simulink model "Hinf_nonlinear_sim"  (R2026a)
settings: Solver=VariableStepAuto
InitFcn:
  | seaDir=fileparts(get_param(bdroot,'FileName'));if isfile(fullfile(seaDir,'..','collaudo_simulink.m')),addpath(fullfile(seaDir,'..'));else,addpath(fullfile(seaDir,'..','..','File_di_Funzioni_Progetto-Accorpati'));end;collaudo_simulink(bdroot);
undefined symbols (not defined in the file): Ak1, Ak2, Bk1, Bk2, Ck1, Ck2, Dk1, Dk2, taubar, xbar
libraries: cstblocks_lti x7
settings Model: Creator=rebec  LastModifiedBy=rebec

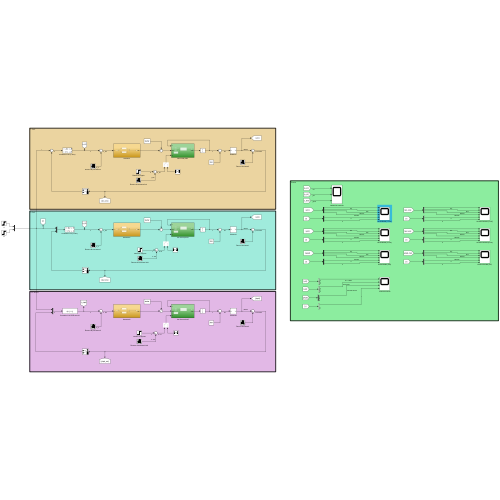
[thumbnail: Simulink's stored preview of the top-level diagram]
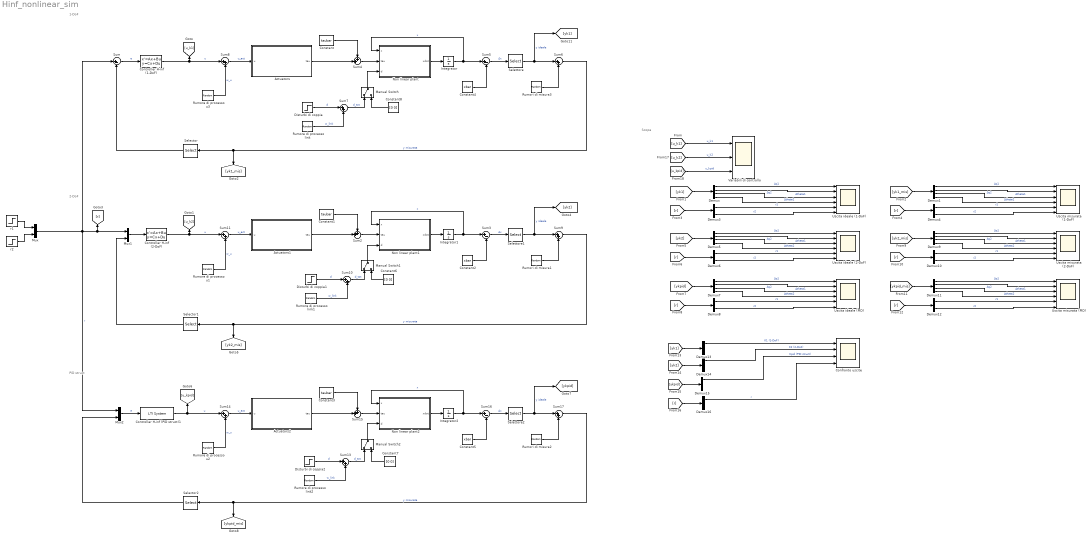
== system Hinf_nonlinear_sim ==
  note: Scope
  note: 2-DoF
  note: PID struct
  note: 1-DoF
  Actuators : Subsystem
  Actuators1 : Subsystem
  Actuators2 : Subsystem
  Confronto uscite : Scope  NumInputPorts=4
      settings: Title=Uscite  ActiveDisplayYMinimum=-0.27933944069600969  ActiveDisplayYMaximum=0.21495071578525782  YLabel=y (rad)  DataLoggingVariableName=ScopeData7
  Constant : Constant  Value=taubar
  Constant1 : Constant  Value=taubar
  Constant2 : Constant  Value=xbar
  Constant3 : Constant  Value=taubar
  Constant4 : Constant  Value=xbar
  Constant5 : Constant  Value=xbar
  Constant6 : Constant  Value=[0 0]
  Constant7 : Constant  Value=[0 0]
  Constant8 : Constant  Value=[0 0]
  Controller H-inf (1-DoF) : StateSpace  A=Ak1  B=Bk1  C=Ck1  D=Dk1  InitialCondition=0
  Controller H-inf (2-DoF) : StateSpace  A=Ak2  B=Bk2  C=Ck2  D=Dk2  InitialCondition=0
  Controller H-inf (PID struct)1 : cstblocks_lti/LTI System  sys=Kpid  IC=[]  PadeOrder=0
      settings: LibrarySourceBlock=cstblocks/LTI System
  Demux{,1,5,7,9,11,13..15} (9 alike) : Demux
  Demux{3..4,6,8,10,12,16} (7 alike) : Demux  Outputs=2
  Disturbi di coppia : Step  Time=[1 1]  InitialValue=[0 0]  FinalValue=[0.5 0]  SampleTime=0
  Disturbi di coppia1 : Step  Time=[1 1]  InitialValue=[0 0]  FinalValue=[0.5 0]  SampleTime=0
  Disturbi di coppia2 : Step  Time=[1 1]  InitialValue=[0 0]  FinalValue=[0.5 0]  SampleTime=0
  Integrator : Integrator  InitialCondition=xbar
  Integrator1 : Integrator  InitialCondition=xbar
  Integrator2 : Integrator  InitialCondition=xbar
  Manual Switch : ManualSwitch
  Manual Switch1 : ManualSwitch
  Manual Switch2 : ManualSwitch
  Mux : Mux  Inputs=2
  Mux1 : Mux  Inputs=2
  Mux2 : Mux  Inputs=2
  Non linear plant : Subsystem
  Non linear plant1 : Subsystem
  Non linear plant2 : Subsystem
  Rumore di processo link : RandomNumber  Mean=[0 0]  Variance=[0.01 0.01]  Seed=20260826  SampleTime=0.002
  Rumore di processo link1 : RandomNumber  Mean=[0 0]  Variance=[0.01 0.01]  Seed=20260826  SampleTime=0.002
  Rumore di processo link2 : RandomNumber  Mean=[0 0]  Variance=[0.01 0.01]  Seed=20260826  SampleTime=0.002
  Rumore di processo u1 : RandomNumber  Mean=[0 0]  Variance=[0.01 0.01]  Seed=20260826  SampleTime=0.002
  Rumore di processo u2 : RandomNumber  Mean=[0 0]  Variance=[0.01 0.01]  Seed=20260826  SampleTime=0.002
  Rumore di processo u3 : RandomNumber  Mean=[0 0]  Variance=[0.01 0.01]  Seed=20260826  SampleTime=0.002
  Rumori di misura1 : RandomNumber  Mean=[0 0 0 0]  Variance=[(0.05*pi/180)^2 (0.05*pi/180)^2 (0.05*pi/180)^2 (0.05*pi/180)^2]  Seed=20260826  SampleTime=0.002
  Rumori di misura2 : RandomNumber  Mean=[0 0 0 0]  Variance=[(0.05*pi/180)^2 (0.05*pi/180)^2 (0.05*pi/180)^2 (0.05*pi/180)^2]  Seed=20260826  SampleTime=0.002
  Rumori di misura3 : RandomNumber  Mean=[0 0 0 0]  Variance=[(0.05*pi/180)^2 (0.05*pi/180)^2 (0.05*pi/180)^2 (0.05*pi/180)^2]  Seed=20260826  SampleTime=0.002
  Selector : Selector  InputPortWidth=4  IndexOptions=Index vector (dialog)  Indices=[1 2]  OutputSizes=1
  Selector1 : Selector  InputPortWidth=4  IndexOptions=Index vector (dialog)  Indices=[1 2]  OutputSizes=1
  Selector2 : Selector  InputPortWidth=4  IndexOptions=Index vector (dialog)  Indices=[1 2]  OutputSizes=1
  Selettore : Selector  InputPortWidth=8  IndexOptions=Index vector (dialog)  Indices=[1 2 5 6]  OutputSizes=1
  Selettore1 : Selector  InputPortWidth=8  IndexOptions=Index vector (dialog)  Indices=[1 2 5 6]  OutputSizes=1
  Selettore2 : Selector  InputPortWidth=8  IndexOptions=Index vector (dialog)  Indices=[1 2 5 6]  OutputSizes=1
  Sum{,3,5,16} (4 alike) : Sum  Inputs=|+-
  Sum{6..11,13..14,17} (9 alike) : Sum  Inputs=|++
  Sum15 : Sum  Inputs=++|
  Sum2 : Sum  Inputs=++|
  Sum4 : Sum  Inputs=++|
  Uscita ideale (1-DoF) : Scope  NumInputPorts=6
      settings: Title=Uscita ideale (1-DoF)  ActiveDisplayYMinimum=-0.57230265617122578  ActiveDisplayYMaximum=0.50667076569906444  YLabel=y (rad)
  Uscita ideale (2-DoF) : Scope  NumInputPorts=6
      settings: Title=Uscita ideale (2-DoF)  ActiveDisplayYMinimum=-0.30624818665705794  ActiveDisplayYMaximum=0.42404349584753864  YLabel=y (rad)  DataLoggingVariableName=ScopeData3
  Uscita ideale (PID) : Scope  NumInputPorts=6
      settings: Title=Uscita ideale (PID struct)  ActiveDisplayYMinimum=-0.20967372209927659  ActiveDisplayYMaximum=0.28461643438199091  YLabel=y (rad)  DataLoggingVariableName=ScopeData4
  Uscita misurata (1-DoF) : Scope  NumInputPorts=6
      settings: Title=Uscita misurata (1-DoF)  ActiveDisplayYMinimum=-0.57230265617122578  ActiveDisplayYMaximum=0.50667076569906444  YLabel=y_m_i_s (rad)
  Uscita misurata (2-DoF) : Scope  NumInputPorts=6
      settings: Title=Uscita misurata (2-DoF)  ActiveDisplayYMinimum=-0.33288828600734088  ActiveDisplayYMaximum=0.43391798062248577  YLabel=y_m_i_s (rad)  DataLoggingVariableName=ScopeData5
  Uscita misurata (PID) : Scope  NumInputPorts=6
      settings: Title=Uscita misurata (PID struct)  ActiveDisplayYMinimum=-0.20967372209927659  ActiveDisplayYMaximum=0.28461643438199091  YLabel=y_m_i_s (rad)  DataLoggingVariableName=ScopeData6
  Variabili di controllo : Scope  NumInputPorts=3
      settings: ActiveDisplayString=3  Title=PID struct  ActiveDisplayYMinimum=-392.20426405655667  ActiveDisplayYMaximum=429.18075042306987  YLabel=u_k_p_i_d (Nm)  DataLoggingVariableName=ScopeData10
  r1 : Step  FinalValue=5*pi/180  SampleTime=0
  r2 : Step  FinalValue=0  SampleTime=0
  wires:
  Demux10/1 -> Uscita misurata (2-DoF)/5  "r1"
  Demux8/1 -> Uscita ideale (PID)/5  "r1"
  Demux8/2 -> Uscita ideale (PID)/6  "r2"
  Demux9/4 -> Uscita misurata (2-DoF)/4  "Δtheta2"
  Demux4/1 -> Uscita misurata (1-DoF)/5  "r1"
  [u_kpid] -> Variabili di controllo/3  "u_kpid"
  Demux15/1 -> Confronto uscite/3  "Kpid (PID struct)"
  r1/1 -> Mux/1
  Demux3/2 -> Uscita ideale (1-DoF)/6  "r2"
  Selector/1 -> Sum/2
  Demux7/3 -> Uscita ideale (PID)/3  "Δtheta1"
  Demux5/3 -> Uscita ideale (2-DoF)/3  "Δtheta1"
  Demux5/2 -> Uscita ideale (2-DoF)/2  "Δq2"
  Demux11/3 -> Uscita misurata (PID)/3  "Δtheta1"
  Demux7/4 -> Uscita ideale (PID)/4  "Δtheta2"
  Demux1/2 -> Uscita misurata (1-DoF)/2  "Δq2"
  Demux1/1 -> Uscita misurata (1-DoF)/1  "Δq1"
  [r] -> Demux10/1
  [yk1_mis] -> Demux1/1
  [r] -> Demux16/1
  [ykpid] -> Demux15/1
  Demux9/2 -> Uscita misurata (2-DoF)/2  "Δq2"
  Controller H-inf (1-DoF)/1 -> Sum8/1, [u_k1]  "u"
  Demux11/4 -> Uscita misurata (PID)/4  "Δtheta2"
  [u_k1] -> Variabili di controllo/1  "u_k1"
  Demux/3 -> Uscita ideale (1-DoF)/3  "Δtheta1"
  Demux11/1 -> Uscita misurata (PID)/1  "Δq1"
  [r] -> Demux3/1
  Demux7/2 -> Uscita ideale (PID)/2  "Δq2"
  Demux/2 -> Uscita ideale (1-DoF)/2  "Δq2"
  Demux9/3 -> Uscita misurata (2-DoF)/3  "Δtheta1"
  [yk2] -> Demux5/1
  [yk2_mis] -> Demux9/1
  Demux14/1 -> Confronto uscite/2  "K2 (2-DoF)"
  [yk1] -> Demux/1
  [ykpid] -> Demux7/1
  Demux5/4 -> Uscita ideale (2-DoF)/4  "Δtheta2"
  Demux/1 -> Uscita ideale (1-DoF)/1  "Δq1"
  r2/1 -> Mux/2
  Demux6/1 -> Uscita ideale (2-DoF)/5  "r1"
  Demux3/1 -> Uscita ideale (1-DoF)/5  "r1"
  Demux4/2 -> Uscita misurata (1-DoF)/6  "r2"
  [r] -> Demux12/1
  [r] -> Demux6/1
  [r] -> Demux8/1
  Demux9/1 -> Uscita misurata (2-DoF)/1  "Δq1"
  Mux/1 -> Mux2/1, Mux1/1, [r], Sum/1  "r"
  Demux1/3 -> Uscita misurata (1-DoF)/3  "Δtheta1"
  Sum/1 -> Controller H-inf (1-DoF)/1  "e"
  Demux13/1 -> Confronto uscite/1  "K1 (1-DoF)"
  Demux6/2 -> Uscita ideale (2-DoF)/6  "r2"
  [yk2] -> Demux14/1
  Demux16/1 -> Confronto uscite/4  "r"
  Demux/4 -> Uscita ideale (1-DoF)/4  "Δtheta2"
  [r] -> Demux4/1
  [yk1] -> Demux13/1
  Demux12/1 -> Uscita misurata (PID)/5  "r1"
  [ykpid_mis] -> Demux11/1
  Demux7/1 -> Uscita ideale (PID)/1  "Δq1"
  Demux5/1 -> Uscita ideale (2-DoF)/1  "Δq1"
  Demux10/2 -> Uscita misurata (2-DoF)/6  "r2"
  Demux1/4 -> Uscita misurata (1-DoF)/4  "Δtheta2"
  Demux11/2 -> Uscita misurata (PID)/2  "Δq2"
  Demux12/2 -> Uscita misurata (PID)/6  "r2"
  [u_k2] -> Variabili di controllo/2  "u_k2"
  Actuators/1(tau) -> Sum4/2
  Disturbi di coppia/1 -> Sum7/1  "d"
  Sum4/1 -> Non linear plant/2(tau)
  Constant/1 -> Sum4/1
  Selettore/1 -> Sum6/1, [yk1]  "y ideale"
  Constant4/1 -> Sum5/2
  Integrator/1 -> Non linear plant/1(x), Sum5/1  "x"
  Sum5/1 -> Selettore/1  "Δx"
  Sum8/1 -> Actuators/1(u)  "u_act"
  Non linear plant/1(xdot) -> Integrator/1
  Sum6/1 -> [yk1_mis], Selector/1  "y misurata"
  Rumore di processo link/1 -> Sum7/2  "w_link"
  Sum9/1 -> [yk2_mis], Selector1/1  "y misurata"
  Controller H-inf (2-DoF)/1 -> Sum11/1, [u_k2]  "u"
  Selector1/1 -> Mux1/2
  Rumore di processo link1/1 -> Sum10/2  "w_link"
  Sum11/1 -> Actuators1/1(u)  "u_act"
  Non linear plant1/1(xdot) -> Integrator1/1
  Sum3/1 -> Selettore1/1  "Δx"
  Selettore1/1 -> Sum9/1, [yk2]  "y ideale"
  Constant2/1 -> Sum3/2
  Sum2/1 -> Non linear plant1/2(tau)
  Integrator1/1 -> Non linear plant1/1(x), Sum3/1  "x"
  Actuators1/1(tau) -> Sum2/2
  Constant1/1 -> Sum2/1
  Disturbi di coppia1/1 -> Sum10/1  "d"
  Constant3/1 -> Sum15/1
  Actuators2/1(tau) -> Sum15/2
  Disturbi di coppia2/1 -> Sum13/1  "d"
  Selettore2/1 -> Sum17/1, [ykpid]  "y ideale"
  Sum15/1 -> Non linear plant2/2(tau)
  Constant5/1 -> Sum16/2
  Mux2/1 -> Controller H-inf (PID struct)1/1  "e"
  Sum16/1 -> Selettore2/1  "Δx"
  Controller H-inf (PID struct)1/1 -> Sum14/1, [u_kpid]  "u"
  Selector2/1 -> Mux2/2
  Rumore di processo link2/1 -> Sum13/2  "w_link"
  Sum14/1 -> Actuators2/1(u)  "u_act"
  Sum17/1 -> [ykpid_mis], Selector2/1  "y misurata"
  Non linear plant2/1(xdot) -> Integrator2/1
  Integrator2/1 -> Non linear plant2/1(x), Sum16/1  "x"
  Mux1/1 -> Controller H-inf (2-DoF)/1
  Manual Switch/1 -> Non linear plant/3(d)
  Sum7/1 -> Manual Switch/1  "d_tot"
  Constant8/1 -> Manual Switch/2
  Manual Switch1/1 -> Non linear plant1/3(d)
  Sum10/1 -> Manual Switch1/1  "d_tot"
  Constant6/1 -> Manual Switch1/2
  Manual Switch2/1 -> Non linear plant2/3(d)
  Sum13/1 -> Manual Switch2/1  "d_tot"
  Constant7/1 -> Manual Switch2/2
  Rumori di misura1/1 -> Sum9/2
  Rumore di processo u1/1 -> Sum11/2  "w_u"
  Rumore di processo u3/1 -> Sum8/2  "w_u"
  Rumori di misura3/1 -> Sum6/2
  Rumore di processo u2/1 -> Sum14/2  "w_u"
  Rumori di misura2/1 -> Sum17/2

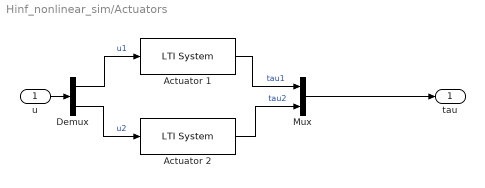
== system Hinf_nonlinear_sim/Actuators ==
  u : Inport
  Actuator 1 : cstblocks_lti/LTI System  sys=Gact  IC=[]  PadeOrder=0
      settings: LibrarySourceBlock=cstblocks/LTI System
  Actuator 2 : cstblocks_lti/LTI System  sys=Gact  IC=[]  PadeOrder=0
      settings: LibrarySourceBlock=cstblocks/LTI System
  Demux : Demux  Outputs=2
  Mux : Mux  Inputs=2
  tau : Outport
  wires:
  Actuator 2/1 -> Mux/2  "tau2"
  Demux/2 -> Actuator 2/1  "u2"
  u/1 -> Demux/1
  Demux/1 -> Actuator 1/1  "u1"
  Mux/1 -> tau/1
  Actuator 1/1 -> Mux/1  "tau1"

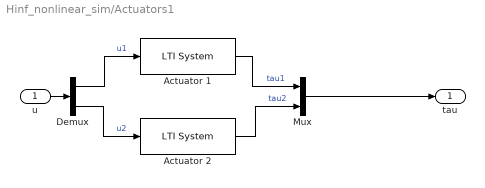
== system Hinf_nonlinear_sim/Actuators1 ==
  u : Inport
  Actuator 1 : cstblocks_lti/LTI System  sys=Gact  IC=[]  PadeOrder=0
      settings: LibrarySourceBlock=cstblocks/LTI System
  Actuator 2 : cstblocks_lti/LTI System  sys=Gact  IC=[]  PadeOrder=0
      settings: LibrarySourceBlock=cstblocks/LTI System
  Demux : Demux  Outputs=2
  Mux : Mux  Inputs=2
  tau : Outport
  wires:
  Actuator 2/1 -> Mux/2  "tau2"
  Demux/2 -> Actuator 2/1  "u2"
  u/1 -> Demux/1
  Demux/1 -> Actuator 1/1  "u1"
  Mux/1 -> tau/1
  Actuator 1/1 -> Mux/1  "tau1"

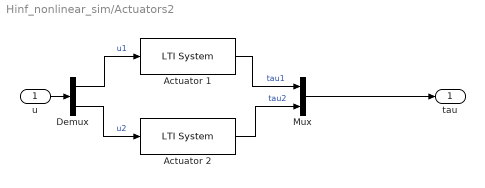
== system Hinf_nonlinear_sim/Actuators2 ==
  u : Inport
  Actuator 1 : cstblocks_lti/LTI System  sys=Gact  IC=[]  PadeOrder=0
      settings: LibrarySourceBlock=cstblocks/LTI System
  Actuator 2 : cstblocks_lti/LTI System  sys=Gact  IC=[]  PadeOrder=0
      settings: LibrarySourceBlock=cstblocks/LTI System
  Demux : Demux  Outputs=2
  Mux : Mux  Inputs=2
  tau : Outport
  wires:
  Actuator 2/1 -> Mux/2  "tau2"
  Demux/2 -> Actuator 2/1  "u2"
  u/1 -> Demux/1
  Demux/1 -> Actuator 1/1  "u1"
  Mux/1 -> tau/1
  Actuator 1/1 -> Mux/1  "tau1"

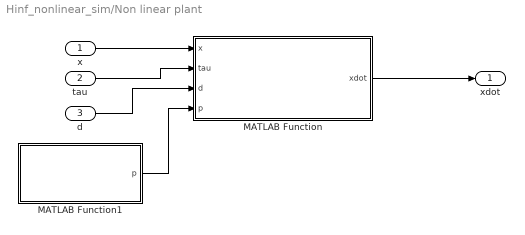
== system Hinf_nonlinear_sim/Non linear plant ==
  x : Inport
  tau : Inport  Port=2
  d : Inport  Port=3
  MATLAB Function : MATLAB Function  TreatAsAtomicUnit=on
  MATLAB Function1 : MATLAB Function  TreatAsAtomicUnit=on
  xdot : Outport
  wires:
  x/1 -> MATLAB Function/1(x)
  tau/1 -> MATLAB Function/2(tau)
  MATLAB Function/1(xdot) -> xdot/1
  MATLAB Function1/1(p) -> MATLAB Function/4(p)
  d/1 -> MATLAB Function/3(d)

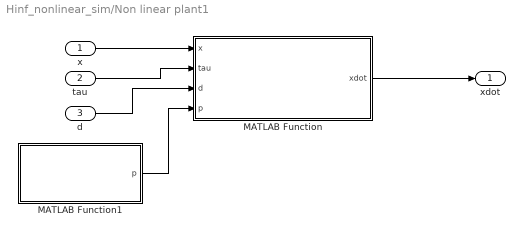
== system Hinf_nonlinear_sim/Non linear plant1 ==
  x : Inport
  tau : Inport  Port=2
  d : Inport  Port=3
  MATLAB Function : MATLAB Function  TreatAsAtomicUnit=on
  MATLAB Function1 : MATLAB Function  TreatAsAtomicUnit=on
  xdot : Outport
  wires:
  x/1 -> MATLAB Function/1(x)
  tau/1 -> MATLAB Function/2(tau)
  MATLAB Function/1(xdot) -> xdot/1
  MATLAB Function1/1(p) -> MATLAB Function/4(p)
  d/1 -> MATLAB Function/3(d)

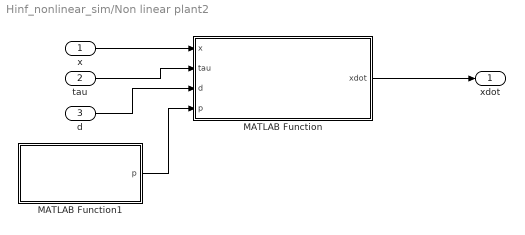
== system Hinf_nonlinear_sim/Non linear plant2 ==
  x : Inport
  tau : Inport  Port=2
  d : Inport  Port=3
  MATLAB Function : MATLAB Function  TreatAsAtomicUnit=on
  MATLAB Function1 : MATLAB Function  TreatAsAtomicUnit=on
  xdot : Outport
  wires:
  x/1 -> MATLAB Function/1(x)
  tau/1 -> MATLAB Function/2(tau)
  MATLAB Function/1(xdot) -> xdot/1
  MATLAB Function1/1(p) -> MATLAB Function/4(p)
  d/1 -> MATLAB Function/3(d)

== matlab function Hinf_nonlinear_sim/Non linear plant/MATLAB Function1 ==
  data: p output Bus: slBus1
function p = sea_params_nominal
%SEA_PARAMS_NOMINAL Nominal mechanical parameters of the 2R SEA robot.
%   P = SEA_PARAMS_NOMINAL returns the values stated by the official
%   assignment. Matrices follow the joint order [joint 1; joint 2].

p.m1 = 1.0;                   % kg
p.m2 = 0.8;                   % kg
p.l1 = 0.4;                   % m
p.l2 = 0.3;                   % m
p.Jm = diag([0.01, 0.01]);    % kg*m^2
p.Bm = diag([0.02, 0.02]);    % N*m*s/rad
p.Ks = diag([50, 40]);        % N*m/rad
p.g = 9.81;                   % m/s^2
end

== matlab function Hinf_nonlinear_sim/Non linear plant/MATLAB Function ==
  data: x input; xdot output; tau input; d input; p input
function xdot = sea_nonlinear_rhs_with_link_disturbance(x, tau, d, p)
%SEA_NONLINEAR_RHS_WITH_LINK_DISTURBANCE SEA dynamics with link torque D.
%   TAU remains the motor-side input; D is an external link-side joint
%   torque entering with positive sign in the link equation.

assert(numel(x) == 8, ...
    'sea_nonlinear_rhs_with_link_disturbance:InvalidState', ...
    'The state must contain exactly eight elements.');
assert(numel(tau) == 2 && numel(d) == 2, ...
    'sea_nonlinear_rhs_with_link_disturbance:InvalidInput', ...
    'Both tau and d must contain exactly two elements.');
x = reshape(x, 8, 1);
tau = reshape(tau, 2, 1);
d = reshape(d, 2, 1);

q = x(1:2);
qdot = x(3:4);
theta = x(5:6);
thetadot = x(7:8);
M = sea_link_inertia(q, p);
C = sea_coriolis(q, qdot, p);
G = sea_gravity(q, p);
tauElastic = sea_elastic_torque(q, theta, p);

qddot = M \ (tauElastic + d - C * qdot - G);
thetaddot = p.Jm \ (tau - p.Bm * thetadot - tauElastic);
xdot = [qdot; qddot; thetadot; thetaddot];
end

== matlab function Hinf_nonlinear_sim/Non linear plant1/MATLAB Function ==
  data: x input; xdot output; tau input; d input; p input
function xdot = sea_nonlinear_rhs_with_link_disturbance(x, tau, d, p)
%SEA_NONLINEAR_RHS_WITH_LINK_DISTURBANCE SEA dynamics with link torque D.
%   TAU remains the motor-side input; D is an external link-side joint
%   torque entering with positive sign in the link equation.

assert(numel(x) == 8, ...
    'sea_nonlinear_rhs_with_link_disturbance:InvalidState', ...
    'The state must contain exactly eight elements.');
assert(numel(tau) == 2 && numel(d) == 2, ...
    'sea_nonlinear_rhs_with_link_disturbance:InvalidInput', ...
    'Both tau and d must contain exactly two elements.');
x = reshape(x, 8, 1);
tau = reshape(tau, 2, 1);
d = reshape(d, 2, 1);

q = x(1:2);
qdot = x(3:4);
theta = x(5:6);
thetadot = x(7:8);
M = sea_link_inertia(q, p);
C = sea_coriolis(q, qdot, p);
G = sea_gravity(q, p);
tauElastic = sea_elastic_torque(q, theta, p);

qddot = M \ (tauElastic + d - C * qdot - G);
thetaddot = p.Jm \ (tau - p.Bm * thetadot - tauElastic);
xdot = [qdot; qddot; thetadot; thetaddot];
end

== matlab function Hinf_nonlinear_sim/Non linear plant1/MATLAB Function1 ==
  data: p output Bus: slBus1
function p = sea_params_nominal
%SEA_PARAMS_NOMINAL Nominal mechanical parameters of the 2R SEA robot.
%   P = SEA_PARAMS_NOMINAL returns the values stated by the official
%   assignment. Matrices follow the joint order [joint 1; joint 2].

p.m1 = 1.0;                   % kg
p.m2 = 0.8;                   % kg
p.l1 = 0.4;                   % m
p.l2 = 0.3;                   % m
p.Jm = diag([0.01, 0.01]);    % kg*m^2
p.Bm = diag([0.02, 0.02]);    % N*m*s/rad
p.Ks = diag([50, 40]);        % N*m/rad
p.g = 9.81;                   % m/s^2
end

== matlab function Hinf_nonlinear_sim/Non linear plant2/MATLAB Function ==
  data: x input; xdot output; tau input; d input; p input
function xdot = sea_nonlinear_rhs_with_link_disturbance(x, tau, d, p)
%SEA_NONLINEAR_RHS_WITH_LINK_DISTURBANCE SEA dynamics with link torque D.
%   TAU remains the motor-side input; D is an external link-side joint
%   torque entering with positive sign in the link equation.

assert(numel(x) == 8, ...
    'sea_nonlinear_rhs_with_link_disturbance:InvalidState', ...
    'The state must contain exactly eight elements.');
assert(numel(tau) == 2 && numel(d) == 2, ...
    'sea_nonlinear_rhs_with_link_disturbance:InvalidInput', ...
    'Both tau and d must contain exactly two elements.');
x = reshape(x, 8, 1);
tau = reshape(tau, 2, 1);
d = reshape(d, 2, 1);

q = x(1:2);
qdot = x(3:4);
theta = x(5:6);
thetadot = x(7:8);
M = sea_link_inertia(q, p);
C = sea_coriolis(q, qdot, p);
G = sea_gravity(q, p);
tauElastic = sea_elastic_torque(q, theta, p);

qddot = M \ (tauElastic + d - C * qdot - G);
thetaddot = p.Jm \ (tau - p.Bm * thetadot - tauElastic);
xdot = [qdot; qddot; thetadot; thetaddot];
end

== matlab function Hinf_nonlinear_sim/Non linear plant2/MATLAB Function1 ==
  data: p output Bus: slBus1
function p = sea_params_nominal
%SEA_PARAMS_NOMINAL Nominal mechanical parameters of the 2R SEA robot.
%   P = SEA_PARAMS_NOMINAL returns the values stated by the official
%   assignment. Matrices follow the joint order [joint 1; joint 2].

p.m1 = 1.0;                   % kg
p.m2 = 0.8;                   % kg
p.l1 = 0.4;                   % m
p.l2 = 0.3;                   % m
p.Jm = diag([0.01, 0.01]);    % kg*m^2
p.Bm = diag([0.02, 0.02]);    % N*m*s/rad
p.Ks = diag([50, 40]);        % N*m/rad
p.g = 9.81;                   % m/s^2
end
